simulink model "online_robot_2024b"  (R2024b)
settings: Solver=FixedStepAuto  StartTime=0.0  StopTime=inf  RelTol=1e-3
undefined symbols (not defined in the file): control_par, controller_index, d, D, is_real_robot, k_theta, k_x, k_y, P_INIT_EKF, q_goal_task1, q_goal_task2, q_init, r, R_2, R_5, R_bad, R_good, T_s, Ts, X, Y
libraries: robotlib x6, simulink x5, sharedtransform x1
(part 2 of 2)

== matlab function online_robot_2024b/localizer/Localizer ==
  data: v input; omega input; Y_vicon input; Ts input; q_est output; q_init input; is_real_robot input; q_pred output
function [q_est, q_pred] = fcn(v, omega, Y_vicon, Ts, q_init, is_real_robot)

    % Extended Kalman Filter with mode-aware initialization
    persistent q_hat P Q initialized
    q_est  = zeros(3,1);
    q_pred = zeros(3,1);
    
    % --- 1. Smart Initialization ---
    if isempty(initialized)
        
        if is_real_robot == 1
            
            % Real robot mode:
            % Wait until valid Vicon data becomes available
            if all(Y_vicon == 0)
                q_est = q_init; % Return initial estimate until data arrives
                q_pred = q_init;
                return;
            else
                q_hat = Y_vicon; % Lock onto the first valid Vicon measurement
                initialized = true;
            end
            
        else
            
            % Simulation mode:
            % Start immediately using q_init
            q_hat = q_init;
            initialized = true;
        end
        
        P = eye(3) * 0.1; 
        
        % Process noise covariance
        % High confidence in odometry model
        Q = diag([1e-4, 1e-4, 5e-4]);
    end

    % --- 2. Prediction Step ---
    
    theta = q_hat(3);
    
    % Nonlinear unicycle kinematic model
    q_pred = zeros(3,1);
    q_pred = q_hat + [v*cos(theta); 
                       v*sin(theta); 
                       omega] * Ts;
                   
    q_pred(3) = wrapToPi(q_pred(3));

    % Jacobian matrix (linearization)
    F = [1, 0, -v*sin(theta)*Ts;
         0, 1,  v*cos(theta)*Ts;
         0, 0,  1];

    P = F * P * F' + Q;

    % --- 3. Update Step ---
    
    % Detect red zone (high sensor noise region)
    in_red = (q_pred(1) >= -0.6 && q_pred(1) <= 0.2);
    
    % Check if Vicon signal is lost
    is_lost = all(Y_vicon == 0);

    if in_red
        
        % High measurement noise covariance inside noisy region
        R = diag([0.7, 0.7, 0.9]);
        
    else
        
        % Low measurement noise covariance in safe region
        R = diag([1e-5, 1e-5, 5e-5]);
    end

    if is_lost
        
        % Task 3:
        % Sensor unavailable, rely only on odometry prediction
        q_est = q_pred;
        
    else
        
        % Standard Kalman Filter update
        
        H = eye(3);
        
        K = (P * H') / (H * P * H' + R);
        
        innovation = Y_vicon - q_pred;
        
        % Correct angular innovation wrapping
        innovation(3) = wrapToPi(innovation(3));
        
        q_est = q_pred + K * innovation;
        q_est(3) = wrapToPi(q_est(3));

        % Covariance update
        P = (eye(3) - K * H) * P;
    end
    
    % Store updated estimate for next iteration
    q_hat = q_est;
end

== matlab function online_robot_2024b/Subsystem1/Subsystem/MATLAB Function ==
  data: u input; y output
function y = manual_unwrap(u)
    % این تابع به صورت دستی عملیات Unwrap را برای سیگنال‌های ورودی انجام می‌دهد.
    
    persistent prev_u cumulative_offset
    
    % مقداردهی اولیه در اولین گام اجرای شبیه‌سازی
    if isempty(prev_u)
        prev_u = u;
        cumulative_offset = zeros(size(u));
    end
    
    % محاسبه اختلاف زاویه فعلی با قبلی
    diff = u - prev_u;
    
    % شناسایی پرش‌های بزرگتر از 180 درجه (pi رادیان)
    for i = 1:length(u)
        if diff(i) > pi
            cumulative_offset(i) = cumulative_offset(i) - 2*pi;
        elseif diff(i) < -pi
            cumulative_offset(i) = cumulative_offset(i) + 2*pi;
        end
    end
    
    % اعمال آفست تجمعی به ورودی فعلی
    y = u + cumulative_offset;
    
    % ذخیره مقدار فعلی برای استفاده در گام بعدی
    prev_u = u;
end

== matlab function online_robot_2024b/DDR ==
  data: u input; omega_wheels output; r parameter; d parameter
function omega_wheels = kin2omegawheels(u, r, d)
omega_l = u(1)/r-d/(2*r)*u(2);
omega_r = u(1)/r+d/(2*r)*u(2);
omega_wheels = [omega_l;omega_r];
% omega_wheels = [omega_r;omega_l];
